simulink model "CorleyLorenz1998_HFI"  (R2024b)
settings: Solver=FixedStepDiscrete  StartTime=0  StopTime=1.1  FixedStep=TsHfi  RelTol=1e-3
InitFcn:
  | demoModel=bdroot; demoWorkspace=get_param(demoModel,'ModelWorkspace');
  | demoCases=getVariable(demoWorkspace,'DemoCases');
  | demoCaseName=get_param([demoModel '/Experiment_Settings'],'CaseName');
  | demoSelected=find(strcmp(demoCaseName,{demoCases.name}),1);
  | demoValues=demoCases(demoSelected).variables; demoNames=fieldnames(demoValues);
  | for demoIndex=1:numel(demoNames), assignin(demoWorkspace,demoNames{demoIndex},demoValues.(demoNames{demoIndex})); end
  | clear demoModel demoWorkspace demoCases demoCaseName demoSelected demoValues demoNames demoIndex;
model workspace (MAT data in the model file):
  BenchTheta = 1.04719758034
  DemoCases : object (value not decoded)
  RecordedSignalNames : object (value not decoded)
  ScenarioData = [0 2.5e-05 5e-05 7.5e-05 0.0001 0.000125 0.00015 0.000175 0.0002 0.000225 0.00025 0.000275 ... (308007 elements, 44001x7)]
values from neighbouring files (symbols this model uses):
  BpfA = 1.0 -1.60953951 0.692369938    [CorleyLorenz1998_HFI.sldd]
  BpfB = 0.153815016 0.0 -0.153815016    [CorleyLorenz1998_HFI.sldd]
  CarrierStep = 0.314159274    [CorleyLorenz1998_HFI.sldd]
  ErrorScale = 6.46270466    [CorleyLorenz1998_HFI.sldd]
  FluxPm = 0.013    [CorleyLorenz1998_HFI.sldd]
  Inertia = 0.0014    [CorleyLorenz1998_HFI.sldd]
  InvCarrierOmega = 7.95774686E-5    [CorleyLorenz1998_HFI.sldd]
  Ld = 0.00045    [CorleyLorenz1998_HFI.sldd]
  LpfA = 1.0 -0.959982038    [CorleyLorenz1998_HFI.sldd]
  LpfB = 0.0400179625    [CorleyLorenz1998_HFI.sldd]
  Lq = 0.0008    [CorleyLorenz1998_HFI.sldd]
  ObsL = 1446628.88    [CorleyLorenz1998_HFI.sldd]
  ObsP = 339.292    [CorleyLorenz1998_HFI.sldd]
  ObsV = 38373.0234    [CorleyLorenz1998_HFI.sldd]
  PolePairs = 2.0    [CorleyLorenz1998_HFI.sldd]
  Rstator = 0.24    [CorleyLorenz1998_HFI.sldd]
  ThetaHatInitial = 0.436332315    [CorleyLorenz1998_HFI.sldd]
  TsHfi = 2.5E-5    [CorleyLorenz1998_HFI.sldd]
  TsSingle = 2.5E-5    [CorleyLorenz1998_HFI.sldd]
  TwoPi = 6.28318548    [CorleyLorenz1998_HFI.sldd]
  Vdc = 48.0    [CorleyLorenz1998_HFI.sldd]
undefined symbols (not defined in the file or in its folder): DiscIntNeverNeededParam
(part 2 of 2)

== system CorleyLorenz1998_HFI/Experiment_Settings ==

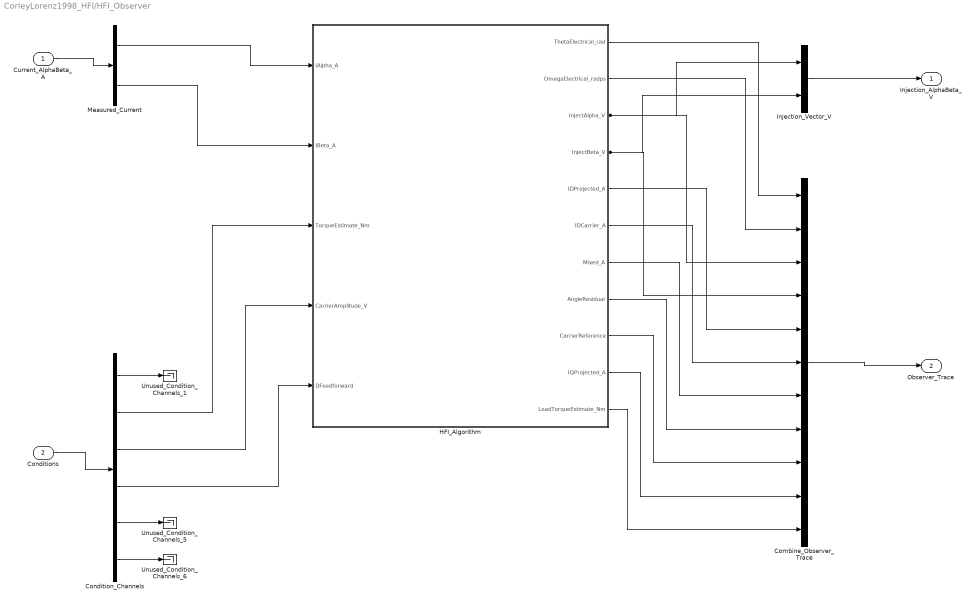
== system CorleyLorenz1998_HFI/HFI_Observer ==
  Current_AlphaBeta_A : Inport
  Conditions : Inport  Port=2
  Combine_Observer_Trace : Mux  Inputs=11
  Condition_Channels : Demux  Outputs=6
  HFI_Algorithm : Subsystem
  Injection_Vector_V : Mux  Inputs=2
  Measured_Current : Demux  Outputs=2
  Unused_Condition_Channels_1 : Terminator
  Unused_Condition_Channels_5 : Terminator
  Unused_Condition_Channels_6 : Terminator
  Injection_AlphaBeta_V : Outport
  Observer_Trace : Outport  Port=2
  wires:
  Combine_Observer_Trace/1 -> Observer_Trace/1
  Injection_Vector_V/1 -> Injection_AlphaBeta_V/1
  HFI_Algorithm/11(LoadTorqueEstimate_Nm) -> Combine_Observer_Trace/11
  HFI_Algorithm/10(IQProjected_A) -> Combine_Observer_Trace/10
  HFI_Algorithm/9(CarrierReference) -> Combine_Observer_Trace/9
  HFI_Algorithm/8(AngleResidual) -> Combine_Observer_Trace/8
  HFI_Algorithm/7(Mixed_A) -> Combine_Observer_Trace/7
  HFI_Algorithm/6(IDCarrier_A) -> Combine_Observer_Trace/6
  HFI_Algorithm/5(IDProjected_A) -> Combine_Observer_Trace/5
  HFI_Algorithm/2(OmegaElectrical_radps) -> Combine_Observer_Trace/2
  HFI_Algorithm/1(ThetaElectrical_rad) -> Combine_Observer_Trace/1
  HFI_Algorithm/4(InjectBeta_V) -> Injection_Vector_V/2, Combine_Observer_Trace/4
  HFI_Algorithm/3(InjectAlpha_V) -> Injection_Vector_V/1, Combine_Observer_Trace/3
  Measured_Current/2 -> HFI_Algorithm/2(IBeta_A)
  Measured_Current/1 -> HFI_Algorithm/1(IAlpha_A)
  Current_AlphaBeta_A/1 -> Measured_Current/1
  Conditions/1 -> Condition_Channels/1
  Condition_Channels/2 -> HFI_Algorithm/3(TorqueEstimate_Nm)
  Condition_Channels/3 -> HFI_Algorithm/4(CarrierAmplitude_V)
  Condition_Channels/4 -> HFI_Algorithm/5(DFeedforward)
  Condition_Channels/1 -> Unused_Condition_Channels_1/1
  Condition_Channels/5 -> Unused_Condition_Channels_5/1
  Condition_Channels/6 -> Unused_Condition_Channels_6/1

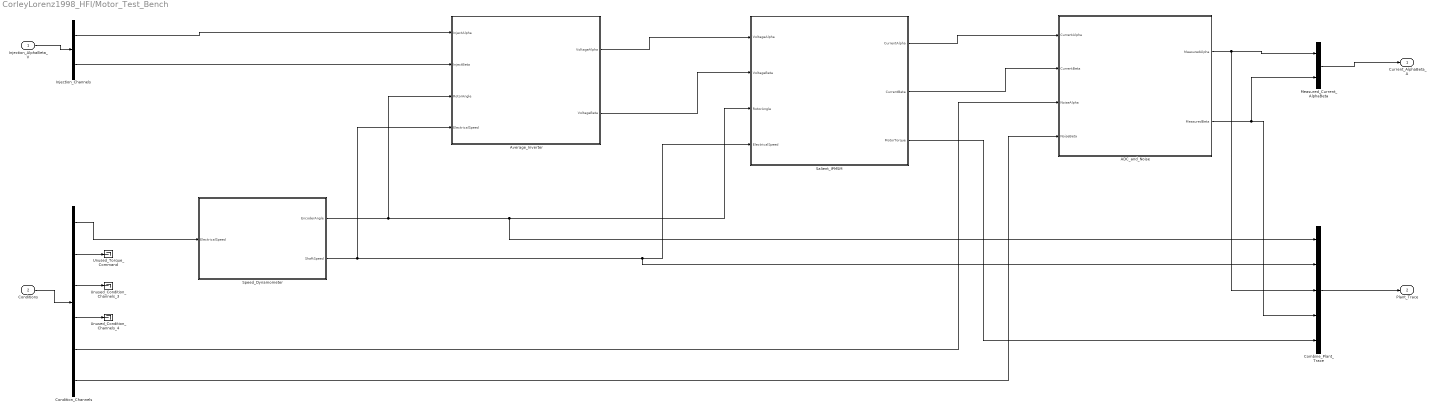
== system CorleyLorenz1998_HFI/Motor_Test_Bench ==
  Injection_AlphaBeta_V : Inport
  Conditions : Inport  Port=2
  ADC_and_Noise : Subsystem
  Average_Inverter : Subsystem
  Combine_Plant_Trace : Mux  Inputs=5
  Condition_Channels : Demux  Outputs=6
  Injection_Channels : Demux  Outputs=2
  Measured_Current_AlphaBeta : Mux  Inputs=2
  Salient_IPMSM : Subsystem
  Speed_Dynamometer : Subsystem
  Unused_Condition_Channels_3 : Terminator
  Unused_Condition_Channels_4 : Terminator
  Unused_Torque_Command : Terminator
  Current_AlphaBeta_A : Outport
  Plant_Trace : Outport  Port=2
  wires:
  Injection_AlphaBeta_V/1 -> Injection_Channels/1
  Conditions/1 -> Condition_Channels/1
  Condition_Channels/1 -> Speed_Dynamometer/1(ElectricalSpeed)
  Condition_Channels/3 -> Unused_Condition_Channels_3/1
  Condition_Channels/4 -> Unused_Condition_Channels_4/1
  Injection_Channels/1 -> Average_Inverter/1(InjectAlpha)
  Speed_Dynamometer/1(EncoderAngle) -> Salient_IPMSM/3(RotorAngle), Combine_Plant_Trace/1, Average_Inverter/3(RotorAngle)
  Average_Inverter/1(VoltageAlpha) -> Salient_IPMSM/1(VoltageAlpha)
  Salient_IPMSM/1(CurrentAlpha) -> ADC_and_Noise/1(CurrentAlpha)
  Condition_Channels/5 -> ADC_and_Noise/3(NoiseAlpha)
  Injection_Channels/2 -> Average_Inverter/2(InjectBeta)
  Speed_Dynamometer/2(ShaftSpeed) -> Salient_IPMSM/4(ElectricalSpeed), Combine_Plant_Trace/2, Average_Inverter/4(ElectricalSpeed)
  Average_Inverter/2(VoltageBeta) -> Salient_IPMSM/2(VoltageBeta)
  Salient_IPMSM/2(CurrentBeta) -> ADC_and_Noise/2(CurrentBeta)
  Condition_Channels/6 -> ADC_and_Noise/4(NoiseBeta)
  ADC_and_Noise/1(MeasuredAlpha) -> Combine_Plant_Trace/3, Measured_Current_AlphaBeta/1
  ADC_and_Noise/2(MeasuredBeta) -> Combine_Plant_Trace/4, Measured_Current_AlphaBeta/2
  Salient_IPMSM/3(MotorTorque) -> Combine_Plant_Trace/5
  Measured_Current_AlphaBeta/1 -> Current_AlphaBeta_A/1
  Combine_Plant_Trace/1 -> Plant_Trace/1
  Condition_Channels/2 -> Unused_Torque_Command/1

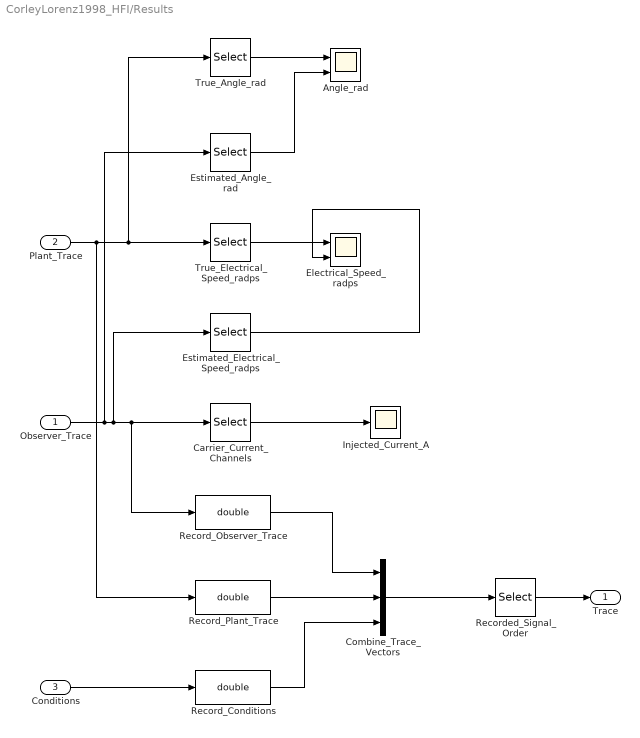
== system CorleyLorenz1998_HFI/Results ==
  Observer_Trace : Inport
  Plant_Trace : Inport  Port=2
  Conditions : Inport  Port=3
  Angle_rad : Scope  NumInputPorts=2
  Carrier_Current_Channels : Selector  InputPortWidth=11  IndexOptions=Index vector (dialog)  Indices=[5 6 10]  OutputSizes=1
  Combine_Trace_Vectors : Mux  Inputs=3
  Electrical_Speed_radps : Scope  NumInputPorts=2
  Estimated_Angle_rad : Selector  InputPortWidth=11  IndexOptions=Index vector (dialog)  Indices=1  OutputSizes=1
  Estimated_Electrical_Speed_radps : Selector  InputPortWidth=11  IndexOptions=Index vector (dialog)  Indices=2  OutputSizes=1
  Injected_Current_A : Scope
  Record_Conditions : DataTypeConversion  OutDataTypeStr=double  SaturateOnIntegerOverflow=off  RndMeth=Floor
  Record_Observer_Trace : DataTypeConversion  OutDataTypeStr=double  SaturateOnIntegerOverflow=off  RndMeth=Floor
  Record_Plant_Trace : DataTypeConversion  OutDataTypeStr=double  SaturateOnIntegerOverflow=off  RndMeth=Floor
  Recorded_Signal_Order : Selector  InputPortWidth=22  IndexOptions=Index vector (dialog)  Indices=[12 13 1:11 14 15 18 19 20 16]  OutputSizes=1
  True_Angle_rad : Selector  InputPortWidth=5  IndexOptions=Index vector (dialog)  Indices=1  OutputSizes=1
  True_Electrical_Speed_radps : Selector  InputPortWidth=5  IndexOptions=Index vector (dialog)  Indices=2  OutputSizes=1
  Trace : Outport
  wires:
  Carrier_Current_Channels/1 -> Injected_Current_A/1
  Estimated_Electrical_Speed_radps/1 -> Electrical_Speed_radps/2
  True_Electrical_Speed_radps/1 -> Electrical_Speed_radps/1
  Estimated_Angle_rad/1 -> Angle_rad/2
  True_Angle_rad/1 -> Angle_rad/1
  Recorded_Signal_Order/1 -> Trace/1
  Combine_Trace_Vectors/1 -> Recorded_Signal_Order/1
  Record_Conditions/1 -> Combine_Trace_Vectors/3
  Record_Plant_Trace/1 -> Combine_Trace_Vectors/2
  Record_Observer_Trace/1 -> Combine_Trace_Vectors/1
  Conditions/1 -> Record_Conditions/1
  Plant_Trace/1 -> True_Angle_rad/1, True_Electrical_Speed_radps/1, Record_Plant_Trace/1
  Observer_Trace/1 -> Record_Observer_Trace/1, Carrier_Current_Channels/1, Estimated_Electrical_Speed_radps/1, Estimated_Angle_rad/1

== system CorleyLorenz1998_HFI/Test_Conditions ==
  Condition_Vector : Mux  Inputs=6
  Scenario_Source : Subsystem
  Conditions : Outport
  wires:
  Condition_Vector/1 -> Conditions/1
  Scenario_Source/6(NoiseBeta) -> Condition_Vector/6
  Scenario_Source/5(NoiseAlpha) -> Condition_Vector/5
  Scenario_Source/4(DComp) -> Condition_Vector/4
  Scenario_Source/3(Amplitude) -> Condition_Vector/3
  Scenario_Source/2(Torque) -> Condition_Vector/2
  Scenario_Source/1(Speed) -> Condition_Vector/1

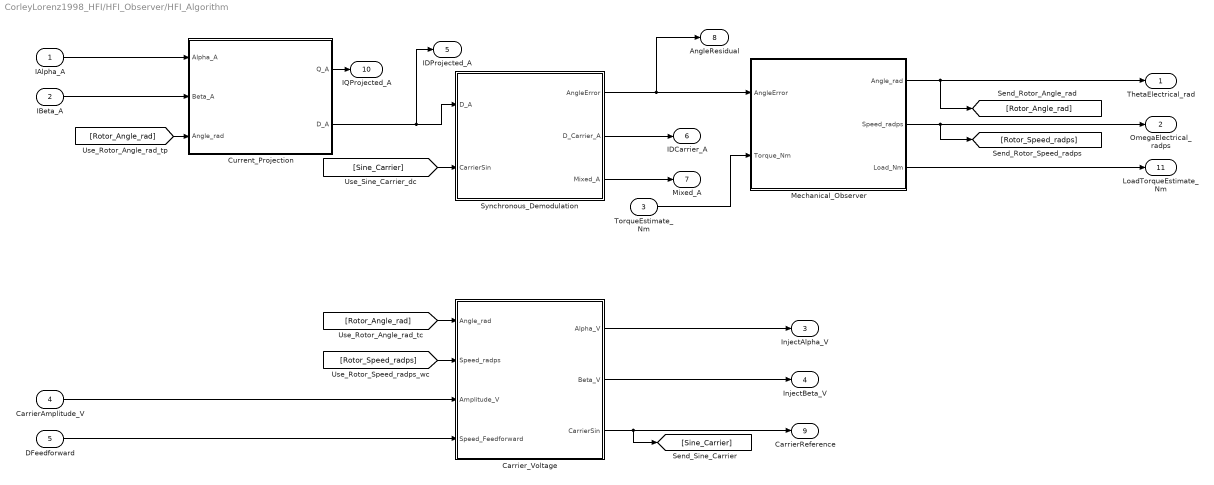
== system CorleyLorenz1998_HFI/HFI_Observer/HFI_Algorithm ==
  IAlpha_A : Inport  OutDataTypeStr=single  SampleTime=TsHfi
  IBeta_A : Inport  Port=2  OutDataTypeStr=single  SampleTime=TsHfi
  TorqueEstimate_Nm : Inport  Port=3  OutDataTypeStr=single  SampleTime=TsHfi
  CarrierAmplitude_V : Inport  Port=4  OutDataTypeStr=single  SampleTime=TsHfi
  DFeedforward : Inport  Port=5  OutDataTypeStr=single  SampleTime=TsHfi
  Carrier_Voltage : Subsystem
  Current_Projection : Subsystem
  Mechanical_Observer : Subsystem
  Synchronous_Demodulation : Subsystem
  ThetaElectrical_rad : Outport
  OmegaElectrical_radps : Outport  Port=2
  InjectAlpha_V : Outport  Port=3
  InjectBeta_V : Outport  Port=4
  IDProjected_A : Outport  Port=5
  IDCarrier_A : Outport  Port=6
  Mixed_A : Outport  Port=7
  AngleResidual : Outport  Port=8
  CarrierReference : Outport  Port=9
  IQProjected_A : Outport  Port=10
  LoadTorqueEstimate_Nm : Outport  Port=11
  wires:
  IAlpha_A/1 -> Current_Projection/1(Alpha_A)
  IBeta_A/1 -> Current_Projection/2(Beta_A)
  [Rotor_Angle_rad] -> Current_Projection/3(Angle_rad)
  Current_Projection/2(D_A) -> IDProjected_A/1, Synchronous_Demodulation/1(D_A)
  Current_Projection/1(Q_A) -> IQProjected_A/1
  [Sine_Carrier] -> Synchronous_Demodulation/2(CarrierSin)
  Synchronous_Demodulation/1(AngleError) -> AngleResidual/1, Mechanical_Observer/1(AngleError)
  Synchronous_Demodulation/2(D_Carrier_A) -> IDCarrier_A/1
  Synchronous_Demodulation/3(Mixed_A) -> Mixed_A/1
  TorqueEstimate_Nm/1 -> Mechanical_Observer/2(Torque_Nm)
  Mechanical_Observer/1(Angle_rad) -> [Rotor_Angle_rad], ThetaElectrical_rad/1
  Mechanical_Observer/2(Speed_radps) -> [Rotor_Speed_radps], OmegaElectrical_radps/1
  Mechanical_Observer/3(Load_Nm) -> LoadTorqueEstimate_Nm/1
  [Rotor_Angle_rad] -> Carrier_Voltage/1(Angle_rad)
  [Rotor_Speed_radps] -> Carrier_Voltage/2(Speed_radps)
  CarrierAmplitude_V/1 -> Carrier_Voltage/3(Amplitude_V)
  DFeedforward/1 -> Carrier_Voltage/4(Speed_Feedforward)
  Carrier_Voltage/1(Alpha_V) -> InjectAlpha_V/1
  Carrier_Voltage/2(Beta_V) -> InjectBeta_V/1
  Carrier_Voltage/3(CarrierSin) -> [Sine_Carrier], CarrierReference/1

== system CorleyLorenz1998_HFI/Motor_Test_Bench/ADC_and_Noise ==
  CurrentAlpha : Inport
  CurrentBeta : Inport  Port=2
  NoiseAlpha : Inport  Port=3
  NoiseBeta : Inport  Port=4
  Alpha_Sample_Plus_Noise : Sum
  Beta_Sample_Plus_Noise : Sum
  MeasuredAlpha : Outport
  MeasuredBeta : Outport  Port=2
  wires:
  Beta_Sample_Plus_Noise/1 -> MeasuredBeta/1
  Alpha_Sample_Plus_Noise/1 -> MeasuredAlpha/1
  NoiseBeta/1 -> Beta_Sample_Plus_Noise/2
  CurrentBeta/1 -> Beta_Sample_Plus_Noise/1
  NoiseAlpha/1 -> Alpha_Sample_Plus_Noise/2
  CurrentAlpha/1 -> Alpha_Sample_Plus_Noise/1

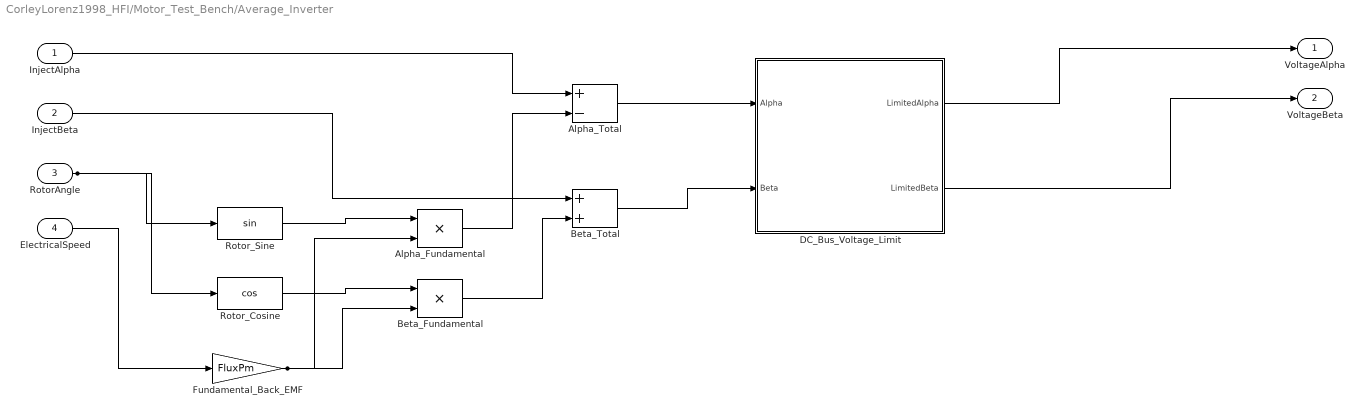
== system CorleyLorenz1998_HFI/Motor_Test_Bench/Average_Inverter ==
  InjectAlpha : Inport
  InjectBeta : Inport  Port=2
  RotorAngle : Inport  Port=3
  ElectricalSpeed : Inport  Port=4
  Alpha_Fundamental : Product  Inputs=**
  Alpha_Total : Sum  Inputs=+-
  Beta_Fundamental : Product  Inputs=**
  Beta_Total : Sum
  DC_Bus_Voltage_Limit : Subsystem
  Fundamental_Back_EMF : Gain  Gain=FluxPm
  Rotor_Cosine : Trigonometry  Operator=cos
  Rotor_Sine : Trigonometry
  VoltageAlpha : Outport
  VoltageBeta : Outport  Port=2
  wires:
  DC_Bus_Voltage_Limit/2(LimitedBeta) -> VoltageBeta/1
  DC_Bus_Voltage_Limit/1(LimitedAlpha) -> VoltageAlpha/1
  Beta_Total/1 -> DC_Bus_Voltage_Limit/2(Beta)
  Alpha_Total/1 -> DC_Bus_Voltage_Limit/1(Alpha)
  Beta_Fundamental/1 -> Beta_Total/2
  InjectBeta/1 -> Beta_Total/1
  Alpha_Fundamental/1 -> Alpha_Total/2
  InjectAlpha/1 -> Alpha_Total/1
  Rotor_Cosine/1 -> Beta_Fundamental/1
  Fundamental_Back_EMF/1 -> Alpha_Fundamental/2, Beta_Fundamental/2
  Rotor_Sine/1 -> Alpha_Fundamental/1
  ElectricalSpeed/1 -> Fundamental_Back_EMF/1
  RotorAngle/1 -> Rotor_Sine/1, Rotor_Cosine/1

== system CorleyLorenz1998_HFI/Motor_Test_Bench/Salient_IPMSM ==
  VoltageAlpha : Inport
  VoltageBeta : Inport  Port=2
  RotorAngle : Inport  Port=3
  ElectricalSpeed : Inport  Port=4
  Current_Inverse_Park : Subsystem
  DQ_Electrical_and_Torque : Subsystem
  Rotor_Cosine : Trigonometry  Operator=cos
  Rotor_Sine : Trigonometry
  Voltage_Park : Subsystem
  CurrentAlpha : Outport
  CurrentBeta : Outport  Port=2
  MotorTorque : Outport  Port=3
  wires:
  DQ_Electrical_and_Torque/3(Torque) -> MotorTorque/1
  Current_Inverse_Park/2(Beta) -> CurrentBeta/1
  Current_Inverse_Park/1(Alpha) -> CurrentAlpha/1
  Rotor_Sine/1 -> Current_Inverse_Park/4(Sin)
  Rotor_Cosine/1 -> Current_Inverse_Park/3(Cos)
  DQ_Electrical_and_Torque/2(Iq) -> Current_Inverse_Park/2(Q)
  DQ_Electrical_and_Torque/1(Id) -> Current_Inverse_Park/1(D)
  ElectricalSpeed/1 -> DQ_Electrical_and_Torque/3(Omega)
  Voltage_Park/1(Q_V) -> DQ_Electrical_and_Torque/2(Vq)
  Voltage_Park/2(D_V) -> DQ_Electrical_and_Torque/1(Vd)
  VoltageBeta/1 -> Voltage_Park/2(Beta_V)
  VoltageAlpha/1 -> Voltage_Park/1(Alpha_V)
  RotorAngle/1 -> Rotor_Cosine/1, Rotor_Sine/1, Voltage_Park/3(Angle_rad)

== system CorleyLorenz1998_HFI/Motor_Test_Bench/Speed_Dynamometer ==
  ElectricalSpeed : Inport
  Encoder_Position : Subsystem
  EncoderAngle : Outport
  ShaftSpeed : Outport  Port=2
  wires:
  Encoder_Position/1(State) -> EncoderAngle/1
  ElectricalSpeed/1 -> Encoder_Position/1(Rate), ShaftSpeed/1

== system CorleyLorenz1998_HFI/Test_Conditions/Scenario_Source ==
  Command_Channels : Demux  Outputs=6
  Shared_Experiment : FromWorkspace  VariableName=ScenarioData  SampleTime=TsHfi  Interpolate=off  OutputAfterFinalValue=Holding final value
  Single_Precision : DataTypeConversion  OutDataTypeStr=single  SaturateOnIntegerOverflow=off  RndMeth=Floor
  Speed : Outport
  Torque : Outport  Port=2
  Amplitude : Outport  Port=3
  DComp : Outport  Port=4
  NoiseAlpha : Outport  Port=5
  NoiseBeta : Outport  Port=6
  wires:
  Command_Channels/6 -> NoiseBeta/1
  Command_Channels/5 -> NoiseAlpha/1
  Command_Channels/4 -> DComp/1
  Command_Channels/3 -> Amplitude/1
  Command_Channels/2 -> Torque/1
  Command_Channels/1 -> Speed/1
  Single_Precision/1 -> Command_Channels/1
  Shared_Experiment/1 -> Single_Precision/1

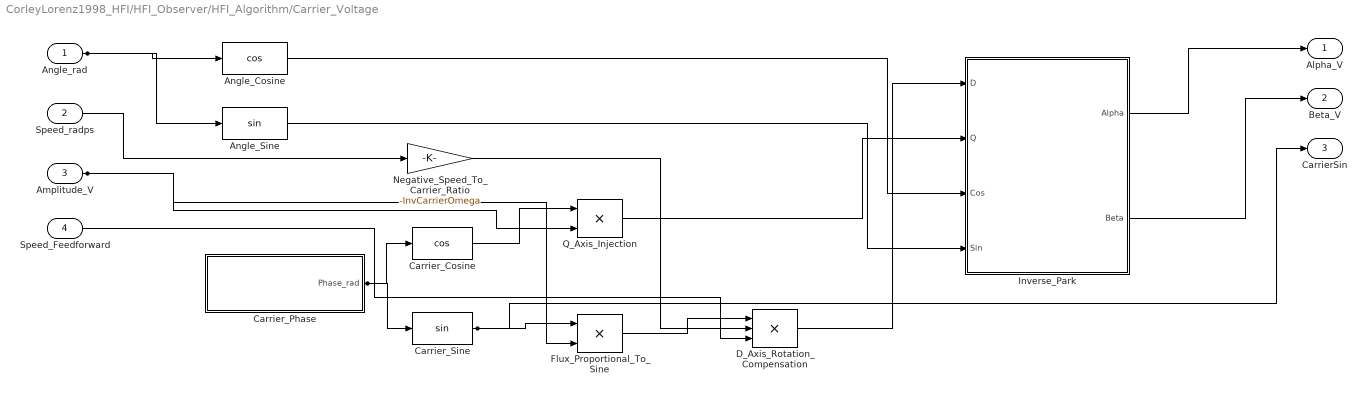
== system CorleyLorenz1998_HFI/HFI_Observer/HFI_Algorithm/Carrier_Voltage ==
  Angle_rad : Inport
  Speed_radps : Inport  Port=2
  Amplitude_V : Inport  Port=3
  Speed_Feedforward : Inport  Port=4
  Angle_Cosine : Trigonometry  Operator=cos
  Angle_Sine : Trigonometry
  Carrier_Cosine : Trigonometry  Operator=cos
  Carrier_Phase : Subsystem
  Carrier_Sine : Trigonometry
  D_Axis_Rotation_Compensation : Product  Inputs=***
  Flux_Proportional_To_Sine : Product  Inputs=**
  Inverse_Park : Subsystem
  Negative_Speed_To_Carrier_Ratio : Gain  Gain=-InvCarrierOmega
  Q_Axis_Injection : Product  Inputs=**
  Alpha_V : Outport
  Beta_V : Outport  Port=2
  CarrierSin : Outport  Port=3
  wires:
  Angle_rad/1 -> Angle_Sine/1, Angle_Cosine/1
  Speed_radps/1 -> Negative_Speed_To_Carrier_Ratio/1
  Carrier_Phase/1(Phase_rad) -> Carrier_Sine/1, Carrier_Cosine/1
  Carrier_Cosine/1 -> Q_Axis_Injection/1
  Amplitude_V/1 -> Flux_Proportional_To_Sine/2, Q_Axis_Injection/2
  Carrier_Sine/1 -> CarrierSin/1, Flux_Proportional_To_Sine/1
  Flux_Proportional_To_Sine/1 -> D_Axis_Rotation_Compensation/1
  Negative_Speed_To_Carrier_Ratio/1 -> D_Axis_Rotation_Compensation/2
  Speed_Feedforward/1 -> D_Axis_Rotation_Compensation/3
  D_Axis_Rotation_Compensation/1 -> Inverse_Park/1(D)
  Q_Axis_Injection/1 -> Inverse_Park/2(Q)
  Angle_Cosine/1 -> Inverse_Park/3(Cos)
  Angle_Sine/1 -> Inverse_Park/4(Sin)
  Inverse_Park/1(Alpha) -> Alpha_V/1
  Inverse_Park/2(Beta) -> Beta_V/1

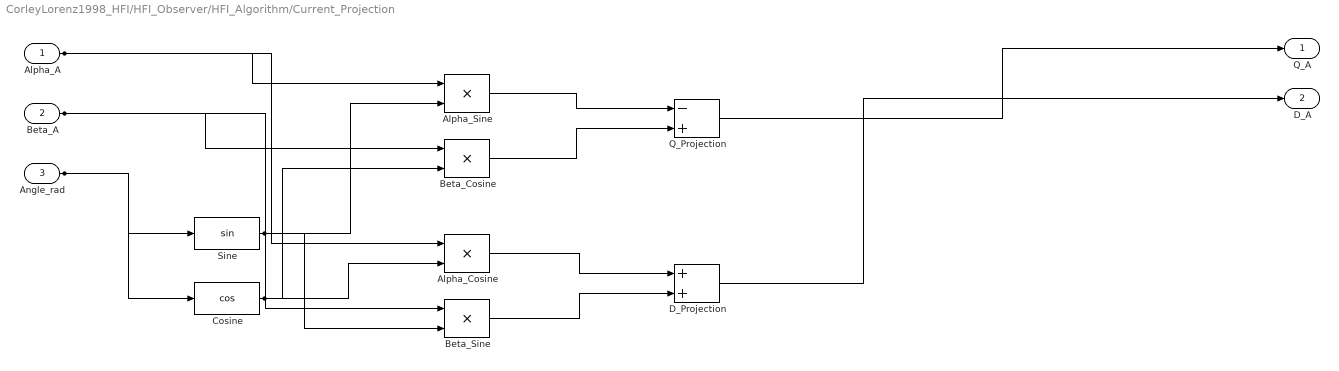
== system CorleyLorenz1998_HFI/HFI_Observer/HFI_Algorithm/Current_Projection ==
  Alpha_A : Inport
  Beta_A : Inport  Port=2
  Angle_rad : Inport  Port=3
  Alpha_Cosine : Product  Inputs=**
  Alpha_Sine : Product  Inputs=**
  Beta_Cosine : Product  Inputs=**
  Beta_Sine : Product  Inputs=**
  Cosine : Trigonometry  Operator=cos
  D_Projection : Sum
  Q_Projection : Sum  Inputs=-+
  Sine : Trigonometry
  Q_A : Outport
  D_A : Outport  Port=2
  wires:
  Angle_rad/1 -> Cosine/1, Sine/1
  Alpha_A/1 -> Alpha_Sine/1, Alpha_Cosine/1
  Sine/1 -> Beta_Sine/2, Alpha_Sine/2
  Beta_A/1 -> Beta_Sine/1, Beta_Cosine/1
  Cosine/1 -> Alpha_Cosine/2, Beta_Cosine/2
  Alpha_Sine/1 -> Q_Projection/1
  Beta_Cosine/1 -> Q_Projection/2
  Alpha_Cosine/1 -> D_Projection/1
  Beta_Sine/1 -> D_Projection/2
  Q_Projection/1 -> Q_A/1
  D_Projection/1 -> D_A/1

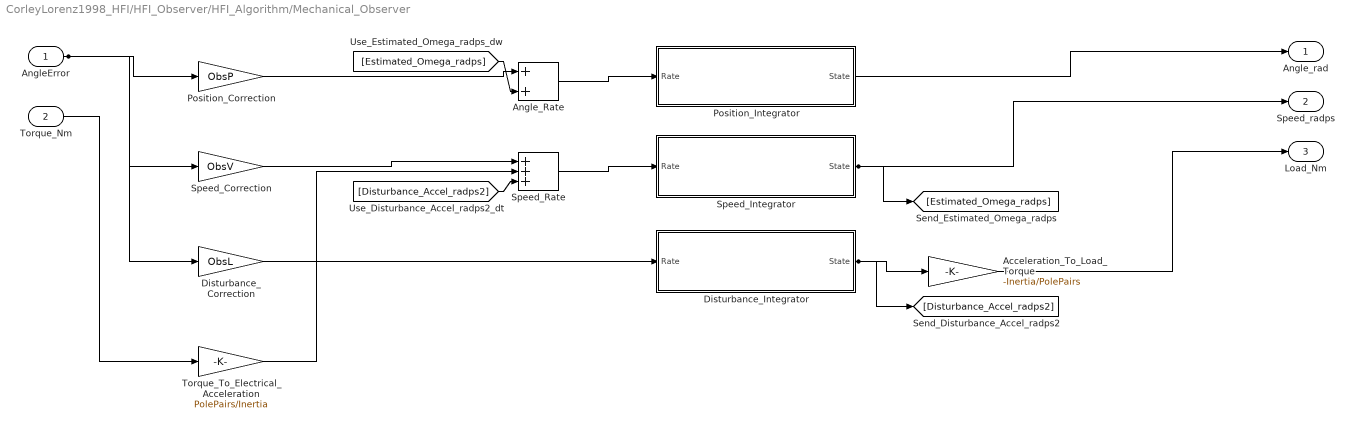
== system CorleyLorenz1998_HFI/HFI_Observer/HFI_Algorithm/Mechanical_Observer ==
  AngleError : Inport
  Torque_Nm : Inport  Port=2
  Acceleration_To_Load_Torque : Gain  Gain=-Inertia/PolePairs
  Angle_Rate : Sum
  Disturbance_Correction : Gain  Gain=ObsL
  Disturbance_Integrator : Subsystem
  Position_Correction : Gain  Gain=ObsP
  Position_Integrator : Subsystem
  Speed_Correction : Gain  Gain=ObsV
  Speed_Integrator : Subsystem
  Speed_Rate : Sum  Inputs=+++
  Torque_To_Electrical_Acceleration : Gain  Gain=PolePairs/Inertia
  Angle_rad : Outport
  Speed_radps : Outport  Port=2
  Load_Nm : Outport  Port=3
  wires:
  AngleError/1 -> Speed_Correction/1, Position_Correction/1, Disturbance_Correction/1
  Torque_Nm/1 -> Torque_To_Electrical_Acceleration/1
  Position_Correction/1 -> Angle_Rate/1
  [Estimated_Omega_radps] -> Angle_Rate/2
  Speed_Correction/1 -> Speed_Rate/1
  Torque_To_Electrical_Acceleration/1 -> Speed_Rate/2
  [Disturbance_Accel_radps2] -> Speed_Rate/3
  Angle_Rate/1 -> Position_Integrator/1(Rate)
  Speed_Rate/1 -> Speed_Integrator/1(Rate)
  Disturbance_Correction/1 -> Disturbance_Integrator/1(Rate)
  Position_Integrator/1(State) -> Angle_rad/1
  Speed_Integrator/1(State) -> Speed_radps/1, [Estimated_Omega_radps]
  Disturbance_Integrator/1(State) -> [Disturbance_Accel_radps2], Acceleration_To_Load_Torque/1
  Acceleration_To_Load_Torque/1 -> Load_Nm/1

== system CorleyLorenz1998_HFI/HFI_Observer/HFI_Algorithm/Synchronous_Demodulation ==
  D_A : Inport
  CarrierSin : Inport  Port=2
  Bandpass_2kHz : DiscreteTransferFcn  Numerator=BpfB  Denominator=BpfA  SampleTime=TsHfi
  Baseband_Lowpass : DiscreteTransferFcn  Numerator=LpfB  Denominator=LpfA  SampleTime=TsHfi
  Multiply_By_Reference : Product  Inputs=**
  Normalize_Small_Angle : Gain  Gain=ErrorScale
  AngleError : Outport
  D_Carrier_A : Outport  Port=2
  Mixed_A : Outport  Port=3
  wires:
  D_A/1 -> Bandpass_2kHz/1
  Bandpass_2kHz/1 -> D_Carrier_A/1, Multiply_By_Reference/1
  CarrierSin/1 -> Multiply_By_Reference/2
  Multiply_By_Reference/1 -> Mixed_A/1, Baseband_Lowpass/1
  Baseband_Lowpass/1 -> Normalize_Small_Angle/1
  Normalize_Small_Angle/1 -> AngleError/1

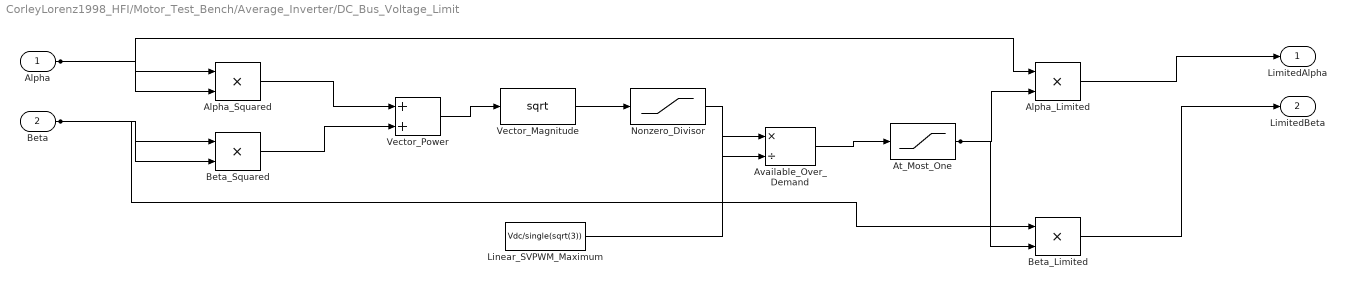
== system CorleyLorenz1998_HFI/Motor_Test_Bench/Average_Inverter/DC_Bus_Voltage_Limit ==
  Alpha : Inport
  Beta : Inport  Port=2
  Alpha_Limited : Product  Inputs=**
  Alpha_Squared : Product  Inputs=**
  At_Most_One : Saturate  UpperLimit=1  LowerLimit=0
  Available_Over_Demand : Product  Inputs=*/
  Beta_Limited : Product  Inputs=**
  Beta_Squared : Product  Inputs=**
  Linear_SVPWM_Maximum : Constant  Value=Vdc/single(sqrt(3))
  Nonzero_Divisor : Saturate  UpperLimit=inf  LowerLimit=single(0.01)
  Vector_Magnitude : Math  Operator=sqrt
  Vector_Power : Sum
  LimitedAlpha : Outport
  LimitedBeta : Outport  Port=2
  wires:
  Beta_Limited/1 -> LimitedBeta/1
  Alpha_Limited/1 -> LimitedAlpha/1
  At_Most_One/1 -> Beta_Limited/2, Alpha_Limited/2
  Available_Over_Demand/1 -> At_Most_One/1
  Nonzero_Divisor/1 -> Available_Over_Demand/2
  Linear_SVPWM_Maximum/1 -> Available_Over_Demand/1
  Vector_Magnitude/1 -> Nonzero_Divisor/1
  Vector_Power/1 -> Vector_Magnitude/1
  Beta_Squared/1 -> Vector_Power/2
  Alpha_Squared/1 -> Vector_Power/1
  Beta/1 -> Beta_Limited/1, Beta_Squared/1, Beta_Squared/2
  Alpha/1 -> Alpha_Limited/1, Alpha_Squared/1, Alpha_Squared/2

== system CorleyLorenz1998_HFI/Motor_Test_Bench/Salient_IPMSM/Current_Inverse_Park ==
  D : Inport
  Q : Inport  Port=2
  Cos : Inport  Port=3
  Sin : Inport  Port=4
  Alpha_Voltage : Sum  Inputs=+-
  Beta_Voltage : Sum
  D_Cosine : Product  Inputs=**
  D_Sine : Product  Inputs=**
  Q_Cosine : Product  Inputs=**
  Q_Sine : Product  Inputs=**
  Alpha : Outport
  Beta : Outport  Port=2
  wires:
  Beta_Voltage/1 -> Beta/1
  Alpha_Voltage/1 -> Alpha/1
  Q_Cosine/1 -> Beta_Voltage/2
  D_Sine/1 -> Beta_Voltage/1
  Q_Sine/1 -> Alpha_Voltage/2
  D_Cosine/1 -> Alpha_Voltage/1
  Sin/1 -> Q_Sine/2, D_Sine/2
  Q/1 -> Q_Sine/1, Q_Cosine/1
  Cos/1 -> D_Cosine/2, Q_Cosine/2
  D/1 -> D_Cosine/1, D_Sine/1

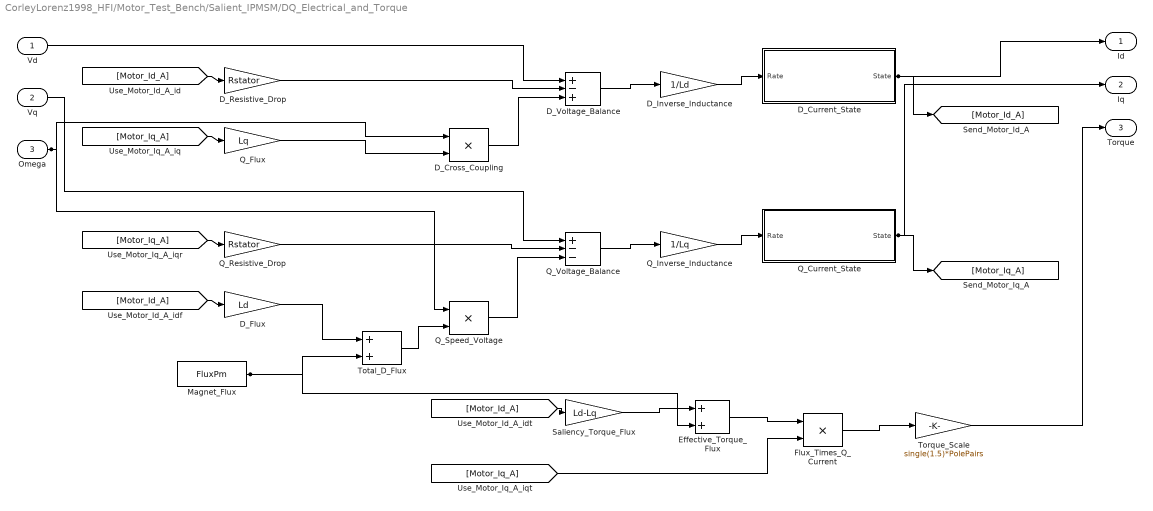
== system CorleyLorenz1998_HFI/Motor_Test_Bench/Salient_IPMSM/DQ_Electrical_and_Torque ==
  Vd : Inport
  Vq : Inport  Port=2
  Omega : Inport  Port=3
  D_Cross_Coupling : Product  Inputs=**
  D_Current_State : Subsystem
  D_Flux : Gain  Gain=Ld
  D_Inverse_Inductance : Gain  Gain=1/Ld
  D_Resistive_Drop : Gain  Gain=Rstator
  D_Voltage_Balance : Sum  Inputs=+-+
  Effective_Torque_Flux : Sum
  Flux_Times_Q_Current : Product  Inputs=**
  Magnet_Flux : Constant  Value=FluxPm
  Q_Current_State : Subsystem
  Q_Flux : Gain  Gain=Lq
  Q_Inverse_Inductance : Gain  Gain=1/Lq
  Q_Resistive_Drop : Gain  Gain=Rstator
  Q_Speed_Voltage : Product  Inputs=**
  Q_Voltage_Balance : Sum  Inputs=+--
  Saliency_Torque_Flux : Gain  Gain=Ld-Lq
  Torque_Scale : Gain  Gain=single(1.5)*PolePairs
  Total_D_Flux : Sum
  Id : Outport
  Iq : Outport  Port=2
  Torque : Outport  Port=3
  wires:
  Torque_Scale/1 -> Torque/1
  Flux_Times_Q_Current/1 -> Torque_Scale/1
  [Motor_Iq_A] -> Flux_Times_Q_Current/2
  Effective_Torque_Flux/1 -> Flux_Times_Q_Current/1
  Saliency_Torque_Flux/1 -> Effective_Torque_Flux/1
  [Motor_Id_A] -> Saliency_Torque_Flux/1
  Q_Current_State/1(State) -> [Motor_Iq_A], Iq/1
  D_Current_State/1(State) -> Id/1, [Motor_Id_A]
  Q_Inverse_Inductance/1 -> Q_Current_State/1(Rate)
  D_Inverse_Inductance/1 -> D_Current_State/1(Rate)
  Q_Voltage_Balance/1 -> Q_Inverse_Inductance/1
  D_Voltage_Balance/1 -> D_Inverse_Inductance/1
  Q_Speed_Voltage/1 -> Q_Voltage_Balance/3
  Q_Resistive_Drop/1 -> Q_Voltage_Balance/2
  Vq/1 -> Q_Voltage_Balance/1
  D_Cross_Coupling/1 -> D_Voltage_Balance/3
  D_Resistive_Drop/1 -> D_Voltage_Balance/2
  Vd/1 -> D_Voltage_Balance/1
  Total_D_Flux/1 -> Q_Speed_Voltage/2
  Q_Flux/1 -> D_Cross_Coupling/2
  Omega/1 -> D_Cross_Coupling/1, Q_Speed_Voltage/1
  Magnet_Flux/1 -> Effective_Torque_Flux/2, Total_D_Flux/2
  D_Flux/1 -> Total_D_Flux/1
  [Motor_Id_A] -> D_Flux/1
  [Motor_Iq_A] -> Q_Resistive_Drop/1
  [Motor_Iq_A] -> Q_Flux/1
  [Motor_Id_A] -> D_Resistive_Drop/1

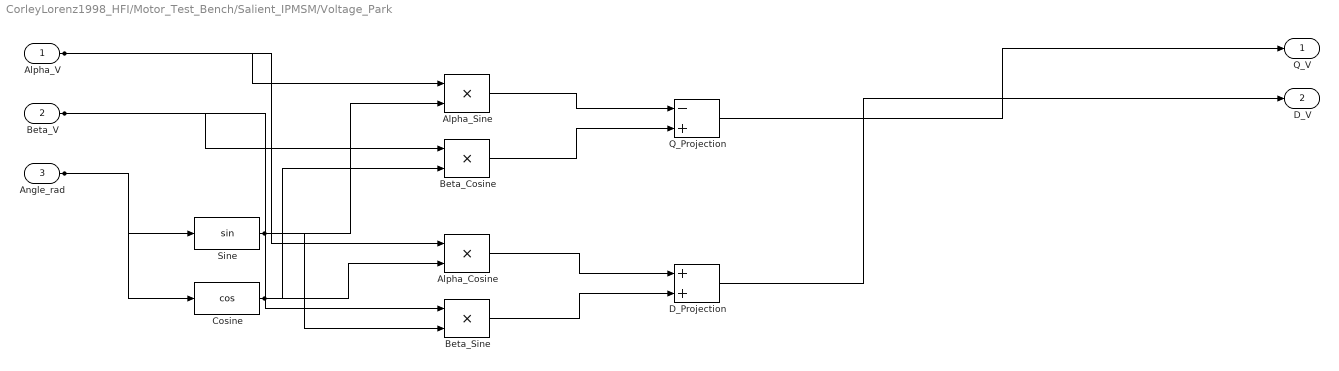
== system CorleyLorenz1998_HFI/Motor_Test_Bench/Salient_IPMSM/Voltage_Park ==
  Alpha_V : Inport
  Beta_V : Inport  Port=2
  Angle_rad : Inport  Port=3
  Alpha_Cosine : Product  Inputs=**
  Alpha_Sine : Product  Inputs=**
  Beta_Cosine : Product  Inputs=**
  Beta_Sine : Product  Inputs=**
  Cosine : Trigonometry  Operator=cos
  D_Projection : Sum
  Q_Projection : Sum  Inputs=-+
  Sine : Trigonometry
  Q_V : Outport
  D_V : Outport  Port=2
  wires:
  D_Projection/1 -> D_V/1
  Q_Projection/1 -> Q_V/1
  Beta_Sine/1 -> D_Projection/2
  Alpha_Cosine/1 -> D_Projection/1
  Beta_Cosine/1 -> Q_Projection/2
  Alpha_Sine/1 -> Q_Projection/1
  Cosine/1 -> Beta_Cosine/2, Alpha_Cosine/2
  Beta_V/1 -> Beta_Cosine/1, Beta_Sine/1
  Sine/1 -> Alpha_Sine/2, Beta_Sine/2
  Alpha_V/1 -> Alpha_Cosine/1, Alpha_Sine/1
  Angle_rad/1 -> Sine/1, Cosine/1

== system CorleyLorenz1998_HFI/Motor_Test_Bench/Speed_Dynamometer/Encoder_Position ==
  Rate : Inport
  Full_Turn : Constant  Value=TwoPi
  Next_State : Sum
  Previous_State : UnitDelay  InitialCondition=BenchTheta  SampleTime=TsHfi  HasFrameUpgradeWarning=on
  Sample_Time : Gain  Gain=TsSingle
  Wrap_To_Turn : Math  Operator=mod
  State : Outport
  wires:
  Wrap_To_Turn/1 -> Previous_State/1
  Next_State/1 -> Wrap_To_Turn/1
  Rate/1 -> Sample_Time/1
  Full_Turn/1 -> Wrap_To_Turn/2
  Previous_State/1 -> Next_State/2, State/1
  Sample_Time/1 -> Next_State/1

== system CorleyLorenz1998_HFI/HFI_Observer/HFI_Algorithm/Carrier_Voltage/Carrier_Phase ==
  Carrier_Step : Constant  Value=CarrierStep
  Full_Turn : Constant  Value=TwoPi
  Next_State : Sum
  Previous_State : UnitDelay  InitialCondition=single(0)  SampleTime=TsHfi  HasFrameUpgradeWarning=on
  Wrap_To_Turn : Math  Operator=mod
  Phase_rad : Outport
  wires:
  Carrier_Step/1 -> Next_State/1
  Previous_State/1 -> Phase_rad/1, Next_State/2
  Full_Turn/1 -> Wrap_To_Turn/2
  Next_State/1 -> Wrap_To_Turn/1
  Wrap_To_Turn/1 -> Previous_State/1

== system CorleyLorenz1998_HFI/HFI_Observer/HFI_Algorithm/Carrier_Voltage/Inverse_Park ==
  D : Inport
  Q : Inport  Port=2
  Cos : Inport  Port=3
  Sin : Inport  Port=4
  Alpha_Voltage : Sum  Inputs=+-
  Beta_Voltage : Sum
  D_Cosine : Product  Inputs=**
  D_Sine : Product  Inputs=**
  Q_Cosine : Product  Inputs=**
  Q_Sine : Product  Inputs=**
  Alpha : Outport
  Beta : Outport  Port=2
  wires:
  D/1 -> D_Sine/1, D_Cosine/1
  Cos/1 -> Q_Cosine/2, D_Cosine/2
  Q/1 -> Q_Cosine/1, Q_Sine/1
  Sin/1 -> D_Sine/2, Q_Sine/2
  D_Cosine/1 -> Alpha_Voltage/1
  Q_Sine/1 -> Alpha_Voltage/2
  D_Sine/1 -> Beta_Voltage/1
  Q_Cosine/1 -> Beta_Voltage/2
  Alpha_Voltage/1 -> Alpha/1
  Beta_Voltage/1 -> Beta/1

== system CorleyLorenz1998_HFI/HFI_Observer/HFI_Algorithm/Mechanical_Observer/Disturbance_Integrator ==
  Rate : Inport
  Next_State : Sum
  Previous_State : UnitDelay  InitialCondition=single(0)  SampleTime=TsHfi  HasFrameUpgradeWarning=on
  Sample_Time : Gain  Gain=TsSingle
  State_Limit : Saturate  UpperLimit=2e5  LowerLimit=-2e5
  State : Outport
  wires:
  Sample_Time/1 -> Next_State/1
  Previous_State/1 -> State/1, Next_State/2
  Rate/1 -> Sample_Time/1
  Next_State/1 -> State_Limit/1
  State_Limit/1 -> Previous_State/1

== system CorleyLorenz1998_HFI/HFI_Observer/HFI_Algorithm/Mechanical_Observer/Position_Integrator ==
  Rate : Inport
  Full_Turn : Constant  Value=TwoPi
  Next_State : Sum
  Previous_State : UnitDelay  InitialCondition=ThetaHatInitial  SampleTime=TsHfi  HasFrameUpgradeWarning=on
  Sample_Time : Gain  Gain=TsSingle
  Wrap_To_Turn : Math  Operator=mod
  State : Outport
  wires:
  Sample_Time/1 -> Next_State/1
  Previous_State/1 -> State/1, Next_State/2
  Full_Turn/1 -> Wrap_To_Turn/2
  Rate/1 -> Sample_Time/1
  Next_State/1 -> Wrap_To_Turn/1
  Wrap_To_Turn/1 -> Previous_State/1

== system CorleyLorenz1998_HFI/HFI_Observer/HFI_Algorithm/Mechanical_Observer/Speed_Integrator ==
  Rate : Inport
  Next_State : Sum
  Previous_State : UnitDelay  InitialCondition=single(0)  SampleTime=TsHfi  HasFrameUpgradeWarning=on
  Sample_Time : Gain  Gain=TsSingle
  State_Limit : Saturate  UpperLimit=1500  LowerLimit=-1500
  State : Outport
  wires:
  Sample_Time/1 -> Next_State/1
  Previous_State/1 -> State/1, Next_State/2
  Rate/1 -> Sample_Time/1
  Next_State/1 -> State_Limit/1
  State_Limit/1 -> Previous_State/1

== system CorleyLorenz1998_HFI/Motor_Test_Bench/Salient_IPMSM/DQ_Electrical_and_Torque/D_Current_State ==
  Rate : Inport
  Forward_Euler : DiscreteIntegrator  InitialCondition=single(0)  SampleTime=TsHfi  ICPrevOutput=DiscIntNeverNeededParam  ICPrevScaledInput=DiscIntNeverNeededParam
  State : Outport
  wires:
  Forward_Euler/1 -> State/1
  Rate/1 -> Forward_Euler/1

== system CorleyLorenz1998_HFI/Motor_Test_Bench/Salient_IPMSM/DQ_Electrical_and_Torque/Q_Current_State ==
  Rate : Inport
  Forward_Euler : DiscreteIntegrator  InitialCondition=single(0)  SampleTime=TsHfi  ICPrevOutput=DiscIntNeverNeededParam  ICPrevScaledInput=DiscIntNeverNeededParam
  State : Outport
  wires:
  Forward_Euler/1 -> State/1
  Rate/1 -> Forward_Euler/1
